simulink model "DWPUSH"  (R2026b)
settings: Solver=VariableStepAuto
undefined symbols (not defined in the file): Ac, Af, Ar, InitLinkage, Left, Linkage, Visual, X, Y, Z
libraries: sm_lib x57, Suspension_Utilities x43, nesl_utility x12, Linkage_Shock x1, fl_lib x1
(part 3 of 4)

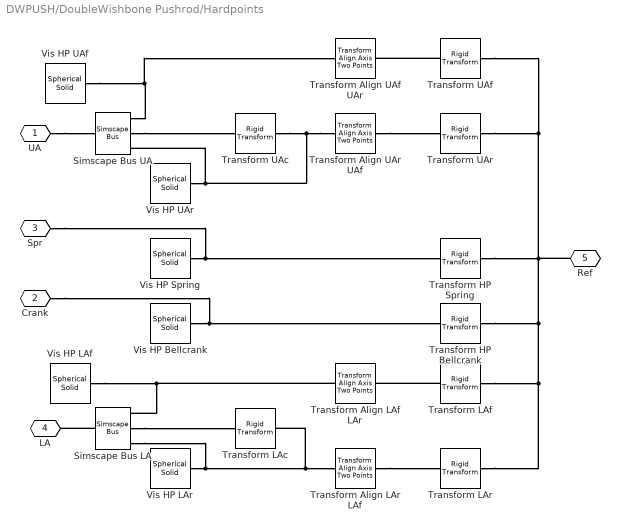
== system DWPUSH/DoubleWishbone Pushrod/Hardpoints ==
  Simscape Bus LA : SimscapeBus  HierarchyStrings=Af;Ac;Ar
  Simscape Bus UA : SimscapeBus  HierarchyStrings=Af;Ac;Ar
  Transform Align LAf LAr : Suspension_Utilities/Transform Align Axis Two Points  hp_b=hp_in_f_la.*rhs_hp  hp_t=hp_in_r_la.*rhs_hp  popup_f_axis=-Z
      settings: SourceProductName=SmCar - Suspension Utilites
  Transform Align LAr LAf : Suspension_Utilities/Transform Align Axis Two Points  hp_b=hp_in_r_la.*rhs_hp  hp_t=hp_in_f_la.*rhs_hp  popup_f_axis=+Z
      settings: SourceProductName=SmCar - Suspension Utilites
  Transform Align UAf UAr : Suspension_Utilities/Transform Align Axis Two Points  hp_b=hp_in_f_ua.*rhs_hp  hp_t=hp_in_r_ua.*rhs_hp  popup_f_axis=-Z
      settings: SourceProductName=SmCar - Suspension Utilites
  Transform Align UAr UAf : Suspension_Utilities/Transform Align Axis Two Points  hp_b=hp_in_r_ua.*rhs_hp  hp_t=hp_in_f_ua.*rhs_hp  popup_f_axis=+Z
      settings: SourceProductName=SmCar - Suspension Utilites
  Transform HP Bellcrank : sm_lib/Frames and Transforms/Rigid Transform  RotationMethod=None  FollAlignAxisA=+X  BaseAlignAxisA=+Y  FollAlignAxisB=+Y  BaseAlignAxisB=+Z  RotationStandardAxis=+Z  RotationAngle=0.0  RotationAngleUnits=deg  RotationArbitraryAxis=[0 0 1]  RotationSequenceAxes=FollowerAxes  RotationSequence=XYX  RotationSequenceAngles=[0 0 0]  RotationSequenceAnglesUnits=deg  RotationMatrix=[1 0 0; 0 1 0; 0 0 1]  Quaternion=[1 0 0 0]  TranslationMethod=Cartesian  TranslationCartesianOffset=hp_bellcrank.*rhs_hp  TranslationCartesianOffsetUnits=m  TranslationStandardAxis=+Z  TranslationStandardOffset=0  TranslationStandardOffsetUnits=m  TranslationROffset=0  TranslationROffsetUnits=m  TranslationThetaOffset=0  TranslationThetaOffsetUnits=deg  TranslationZOffset=0  TranslationZOffsetUnits=m
  Transform HP Spring : sm_lib/Frames and Transforms/Rigid Transform  RotationMethod=None  FollAlignAxisA=+X  BaseAlignAxisA=+Y  FollAlignAxisB=+Y  BaseAlignAxisB=+Z  RotationStandardAxis=+Z  RotationAngle=0.0  RotationAngleUnits=deg  RotationArbitraryAxis=[0 0 1]  RotationSequenceAxes=FollowerAxes  RotationSequence=XYX  RotationSequenceAngles=[0 0 0]  RotationSequenceAnglesUnits=deg  RotationMatrix=[1 0 0; 0 1 0; 0 0 1]  Quaternion=[1 0 0 0]  TranslationMethod=Cartesian  TranslationCartesianOffset=hp_spr_top.*rhs_hp  TranslationCartesianOffsetUnits=m  TranslationStandardAxis=+Z  TranslationStandardOffset=0  TranslationStandardOffsetUnits=m  TranslationROffset=0  TranslationROffsetUnits=m  TranslationThetaOffset=0  TranslationThetaOffsetUnits=deg  TranslationZOffset=0  TranslationZOffsetUnits=m
  Transform LAc : sm_lib/Frames and Transforms/Rigid Transform  RotationMethod=None  FollAlignAxisA=+X  BaseAlignAxisA=+Y  FollAlignAxisB=+Y  BaseAlignAxisB=+Z  RotationStandardAxis=+Z  RotationAngle=0  RotationAngleUnits=deg  RotationArbitraryAxis=[0 0 1]  RotationSequenceAxes=FollowerAxes  RotationSequence=XYX  RotationSequenceAngles=[0 0 0]  RotationSequenceAnglesUnits=deg  RotationMatrix=[0 0 -1;0 1 0;1 0 0]  Quaternion=[1 0 0 0]  TranslationMethod=StandardAxis  TranslationCartesianOffset=[0 0 0]  TranslationCartesianOffsetUnits=m  TranslationStandardAxis=+Z  TranslationStandardOffset=norm(hp_in_f_la-hp_in_r_la)/2  TranslationStandardOffsetUnits=m  TranslationROffset=0  TranslationROffsetUnits=m  TranslationThetaOffset=0  TranslationThetaOffsetUnits=deg  TranslationZOffset=0  TranslationZOffsetUnits=m
  Transform LAf : sm_lib/Frames and Transforms/Rigid Transform  RotationMethod=None  FollAlignAxisA=+X  BaseAlignAxisA=+Y  FollAlignAxisB=+Y  BaseAlignAxisB=+Z  RotationStandardAxis=+Z  RotationAngle=0.0  RotationAngleUnits=deg  RotationArbitraryAxis=[0 0 1]  RotationSequenceAxes=FollowerAxes  RotationSequence=XYX  RotationSequenceAngles=[0 0 0]  RotationSequenceAnglesUnits=deg  RotationMatrix=[1 0 0; 0 1 0; 0 0 1]  Quaternion=[1 0 0 0]  TranslationMethod=Cartesian  TranslationCartesianOffset=hp_in_f_la.*rhs_hp  TranslationCartesianOffsetUnits=m  TranslationStandardAxis=+Z  TranslationStandardOffset=0  TranslationStandardOffsetUnits=m  TranslationROffset=0  TranslationROffsetUnits=m  TranslationThetaOffset=0  TranslationThetaOffsetUnits=deg  TranslationZOffset=0  TranslationZOffsetUnits=m
  Transform LAr : sm_lib/Frames and Transforms/Rigid Transform  RotationMethod=None  FollAlignAxisA=+X  BaseAlignAxisA=+Y  FollAlignAxisB=+Y  BaseAlignAxisB=+Z  RotationStandardAxis=+Z  RotationAngle=0.0  RotationAngleUnits=deg  RotationArbitraryAxis=[0 0 1]  RotationSequenceAxes=FollowerAxes  RotationSequence=XYX  RotationSequenceAngles=[0 0 0]  RotationSequenceAnglesUnits=deg  RotationMatrix=[1 0 0; 0 1 0; 0 0 1]  Quaternion=[1 0 0 0]  TranslationMethod=Cartesian  TranslationCartesianOffset=hp_in_r_la.*rhs_hp  TranslationCartesianOffsetUnits=m  TranslationStandardAxis=+Z  TranslationStandardOffset=0  TranslationStandardOffsetUnits=m  TranslationROffset=0  TranslationROffsetUnits=m  TranslationThetaOffset=0  TranslationThetaOffsetUnits=deg  TranslationZOffset=0  TranslationZOffsetUnits=m
  Transform UAc : sm_lib/Frames and Transforms/Rigid Transform  RotationMethod=None  FollAlignAxisA=+X  BaseAlignAxisA=+Y  FollAlignAxisB=+Y  BaseAlignAxisB=+Z  RotationStandardAxis=+Z  RotationAngle=0  RotationAngleUnits=deg  RotationArbitraryAxis=[0 0 1]  RotationSequenceAxes=FollowerAxes  RotationSequence=XYX  RotationSequenceAngles=[0 0 0]  RotationSequenceAnglesUnits=deg  RotationMatrix=[0 0 -1;0 1 0;1 0 0]  Quaternion=[1 0 0 0]  TranslationMethod=StandardAxis  TranslationCartesianOffset=[0 0 0]  TranslationCartesianOffsetUnits=m  TranslationStandardAxis=+Z  TranslationStandardOffset=norm(hp_in_f_ua - hp_in_r_ua)/2  TranslationStandardOffsetUnits=m  TranslationROffset=0  TranslationROffsetUnits=m  TranslationThetaOffset=0  TranslationThetaOffsetUnits=deg  TranslationZOffset=0  TranslationZOffsetUnits=m
  Transform UAf : sm_lib/Frames and Transforms/Rigid Transform  RotationMethod=None  FollAlignAxisA=+X  BaseAlignAxisA=+Y  FollAlignAxisB=+Y  BaseAlignAxisB=+Z  RotationStandardAxis=+Z  RotationAngle=0.0  RotationAngleUnits=deg  RotationArbitraryAxis=[0 0 1]  RotationSequenceAxes=FollowerAxes  RotationSequence=XYX  RotationSequenceAngles=[0 0 0]  RotationSequenceAnglesUnits=deg  RotationMatrix=[1 0 0; 0 1 0; 0 0 1]  Quaternion=[1 0 0 0]  TranslationMethod=Cartesian  TranslationCartesianOffset=hp_in_f_ua.*rhs_hp  TranslationCartesianOffsetUnits=m  TranslationStandardAxis=+Z  TranslationStandardOffset=0  TranslationStandardOffsetUnits=m  TranslationROffset=0  TranslationROffsetUnits=m  TranslationThetaOffset=0  TranslationThetaOffsetUnits=deg  TranslationZOffset=0  TranslationZOffsetUnits=m
  Transform UAr : sm_lib/Frames and Transforms/Rigid Transform  RotationMethod=None  FollAlignAxisA=+X  BaseAlignAxisA=+Y  FollAlignAxisB=+Y  BaseAlignAxisB=+Z  RotationStandardAxis=+Z  RotationAngle=0.0  RotationAngleUnits=deg  RotationArbitraryAxis=[0 0 1]  RotationSequenceAxes=FollowerAxes  RotationSequence=XYX  RotationSequenceAngles=[0 0 0]  RotationSequenceAnglesUnits=deg  RotationMatrix=[1 0 0; 0 1 0; 0 0 1]  Quaternion=[1 0 0 0]  TranslationMethod=Cartesian  TranslationCartesianOffset=hp_in_r_ua.*rhs_hp  TranslationCartesianOffsetUnits=m  TranslationStandardAxis=+Z  TranslationStandardOffset=0  TranslationStandardOffsetUnits=m  TranslationROffset=0  TranslationROffsetUnits=m  TranslationThetaOffset=0  TranslationThetaOffsetUnits=deg  TranslationZOffset=0  TranslationZOffsetUnits=m
  Vis HP Bellcrank : sm_lib/Body Elements/Spherical Solid  SphereRadius=size_hp  SphereRadiusUnits=m  ExportEntireGeometry=off  InertiaType=CalculateFromGeometry  BasedOnType=Density  Density=0  DensityUnits=kg/m^3  Mass=1  MassUnits=kg  CenterOfMass=[0 0 0]  CenterOfMassUnits=m  MomentsOfInertia=[1 1 1]  MomentsOfInertiaUnits=kg*m^2  ProductsOfInertia=[0 0 0]  ProductsOfInertiaUnits=kg*m^2  GraphicType=FromGeometry  MarkerShape=Sphere  MarkerSize=10  GraphicVisPropType=SimpleVisualProperties  GraphicDiffuseColor=clr_hp  GraphicOpacity=opc_hp  GraphicSpecularColor=[0.5 0.5 0.5 1.0]  GraphicAmbientColor=[0.15 0.15 0.15 1.0]  GraphicEmissiveColor=[0.0 0.0 0.0 1.0]  GraphicShininess=75  DoExposeReferenceFrame=on  SerializedFrames=<Frames/>
  Vis HP LAf : sm_lib/Body Elements/Spherical Solid  SphereRadius=size_hp  SphereRadiusUnits=m  ExportEntireGeometry=off  InertiaType=CalculateFromGeometry  BasedOnType=Density  Density=0  DensityUnits=kg/m^3  Mass=1  MassUnits=kg  CenterOfMass=[0 0 0]  CenterOfMassUnits=m  MomentsOfInertia=[1 1 1]  MomentsOfInertiaUnits=kg*m^2  ProductsOfInertia=[0 0 0]  ProductsOfInertiaUnits=kg*m^2  GraphicType=FromGeometry  MarkerShape=Sphere  MarkerSize=10  GraphicVisPropType=SimpleVisualProperties  GraphicDiffuseColor=clr_hp  GraphicOpacity=opc_hp  GraphicSpecularColor=[0.5 0.5 0.5 1.0]  GraphicAmbientColor=[0.15 0.15 0.15 1.0]  GraphicEmissiveColor=[0.0 0.0 0.0 1.0]  GraphicShininess=75  DoExposeReferenceFrame=on  SerializedFrames=<Frames/>
  Vis HP LAr : sm_lib/Body Elements/Spherical Solid  SphereRadius=size_hp  SphereRadiusUnits=m  ExportEntireGeometry=off  InertiaType=CalculateFromGeometry  BasedOnType=Density  Density=0  DensityUnits=kg/m^3  Mass=1  MassUnits=kg  CenterOfMass=[0 0 0]  CenterOfMassUnits=m  MomentsOfInertia=[1 1 1]  MomentsOfInertiaUnits=kg*m^2  ProductsOfInertia=[0 0 0]  ProductsOfInertiaUnits=kg*m^2  GraphicType=FromGeometry  MarkerShape=Sphere  MarkerSize=10  GraphicVisPropType=SimpleVisualProperties  GraphicDiffuseColor=clr_hp  GraphicOpacity=opc_hp  GraphicSpecularColor=[0.5 0.5 0.5 1.0]  GraphicAmbientColor=[0.15 0.15 0.15 1.0]  GraphicEmissiveColor=[0.0 0.0 0.0 1.0]  GraphicShininess=75  DoExposeReferenceFrame=on  SerializedFrames=<Frames/>
  Vis HP Spring : sm_lib/Body Elements/Spherical Solid  SphereRadius=size_hp  SphereRadiusUnits=m  ExportEntireGeometry=off  InertiaType=CalculateFromGeometry  BasedOnType=Density  Density=0  DensityUnits=kg/m^3  Mass=1  MassUnits=kg  CenterOfMass=[0 0 0]  CenterOfMassUnits=m  MomentsOfInertia=[1 1 1]  MomentsOfInertiaUnits=kg*m^2  ProductsOfInertia=[0 0 0]  ProductsOfInertiaUnits=kg*m^2  GraphicType=FromGeometry  MarkerShape=Sphere  MarkerSize=10  GraphicVisPropType=SimpleVisualProperties  GraphicDiffuseColor=clr_hp  GraphicOpacity=opc_hp  GraphicSpecularColor=[0.5 0.5 0.5 1.0]  GraphicAmbientColor=[0.15 0.15 0.15 1.0]  GraphicEmissiveColor=[0.0 0.0 0.0 1.0]  GraphicShininess=75  DoExposeReferenceFrame=on  SerializedFrames=<Frames/>
  Vis HP UAf : sm_lib/Body Elements/Spherical Solid  SphereRadius=size_hp  SphereRadiusUnits=m  ExportEntireGeometry=off  InertiaType=CalculateFromGeometry  BasedOnType=Density  Density=0  DensityUnits=kg/m^3  Mass=1  MassUnits=kg  CenterOfMass=[0 0 0]  CenterOfMassUnits=m  MomentsOfInertia=[1 1 1]  MomentsOfInertiaUnits=kg*m^2  ProductsOfInertia=[0 0 0]  ProductsOfInertiaUnits=kg*m^2  GraphicType=FromGeometry  MarkerShape=Sphere  MarkerSize=10  GraphicVisPropType=SimpleVisualProperties  GraphicDiffuseColor=clr_hp  GraphicOpacity=opc_hp  GraphicSpecularColor=[0.5 0.5 0.5 1.0]  GraphicAmbientColor=[0.15 0.15 0.15 1.0]  GraphicEmissiveColor=[0.0 0.0 0.0 1.0]  GraphicShininess=75  DoExposeReferenceFrame=on  SerializedFrames=<Frames/>
  Vis HP UAr : sm_lib/Body Elements/Spherical Solid  SphereRadius=size_hp  SphereRadiusUnits=m  ExportEntireGeometry=off  InertiaType=CalculateFromGeometry  BasedOnType=Density  Density=0  DensityUnits=kg/m^3  Mass=1  MassUnits=kg  CenterOfMass=[0 0 0]  CenterOfMassUnits=m  MomentsOfInertia=[1 1 1]  MomentsOfInertiaUnits=kg*m^2  ProductsOfInertia=[0 0 0]  ProductsOfInertiaUnits=kg*m^2  GraphicType=FromGeometry  MarkerShape=Sphere  MarkerSize=10  GraphicVisPropType=SimpleVisualProperties  GraphicDiffuseColor=clr_hp  GraphicOpacity=opc_hp  GraphicSpecularColor=[0.5 0.5 0.5 1.0]  GraphicAmbientColor=[0.15 0.15 0.15 1.0]  GraphicEmissiveColor=[0.0 0.0 0.0 1.0]  GraphicShininess=75  DoExposeReferenceFrame=on  SerializedFrames=<Frames/>
  UA : PMIOPort  Side=Left
  Crank : PMIOPort  Port=2  Side=Left
  Spr : PMIOPort  Port=3  Side=Left
  LA : PMIOPort  Port=4  Side=Left
  Ref : PMIOPort  Port=5  Side=Right
  connections:
  Transform LAf/RConn1 -- Transform Align LAf LAr/LConn1
  Transform Align LAr LAf/LConn1 -- Transform LAr/RConn1
  Transform Align UAr UAf/RConn1 -- Vis HP UAr/RConn1 -- Simscape Bus UA/LConn3 -- Transform UAc/LConn1
  Transform Align UAr UAf/LConn1 -- Transform UAr/RConn1
  Transform UAf/RConn1 -- Transform Align UAf UAr/LConn1
  Vis HP Spring/RConn1 -- Spr/RConn1 -- Transform HP Spring/RConn1
  Simscape Bus UA/LConn1 -- Vis HP UAf/RConn1 -- Transform Align UAf UAr/RConn1
  Vis HP LAr/RConn1 -- Transform Align LAr LAf/RConn1 -- Transform LAc/LConn1 -- Simscape Bus LA/LConn3
  Vis HP LAf/RConn1 -- Transform Align LAf LAr/RConn1 -- Simscape Bus LA/LConn1
  Ref/RConn1 -- Transform HP Spring/LConn1 -- Transform UAr/LConn1 -- Transform UAf/LConn1 -- Transform HP Bellcrank/LConn1 -- Transform LAf/LConn1 -- Transform LAr/LConn1
  Simscape Bus UA/LConn2 -- Transform UAc/RConn1
  UA/RConn1 -- Simscape Bus UA/RConn1
  Simscape Bus LA/LConn2 -- Transform LAc/RConn1
  Simscape Bus LA/RConn1 -- LA/RConn1
  Vis HP Bellcrank/RConn1 -- Crank/RConn1 -- Transform HP Bellcrank/RConn1

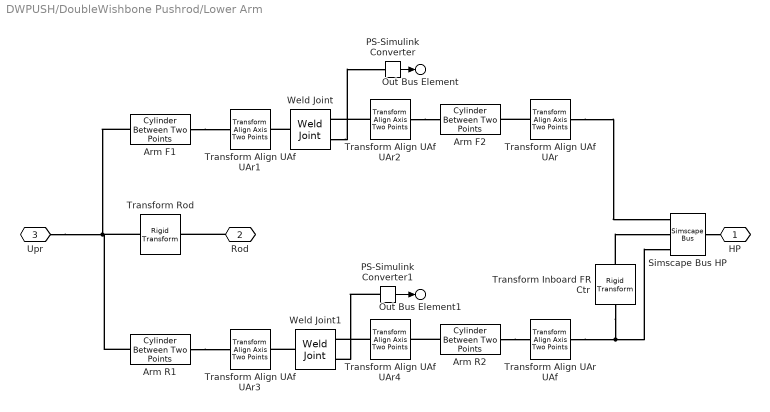
== system DWPUSH/DoubleWishbone Pushrod/Lower Arm ==
  Arm F1 : Suspension_Utilities/Cylinder Between Two Points  hp_b=hp_rod_f.*rhs_hp  hp_f=hp_out.*rhs_hp  Mass=la_mass/2  clr_solid=clr_solid  opc_solid=opc_solid  rad_solid=rad_solid
      settings: SourceProductName=SmCar - Suspension Utilites
  Arm F2 : Suspension_Utilities/Cylinder Between Two Points  hp_b=hp_rod_f.*rhs_hp  hp_f=hp_out.*rhs_hp  Mass=la_mass/2  clr_solid=clr_solid  opc_solid=opc_solid  rad_solid=rad_solid
      settings: SourceProductName=SmCar - Suspension Utilites
  Arm R1 : Suspension_Utilities/Cylinder Between Two Points  hp_b=hp_rod_r.*rhs_hp  hp_f=hp_out.*rhs_hp  Mass=ua_mass/4  clr_solid=clr_solid  opc_solid=opc_solid  rad_solid=rad_solid
      settings: SourceProductName=SmCar - Suspension Utilites
  Arm R2 : Suspension_Utilities/Cylinder Between Two Points  hp_b=hp_in_r.*rhs_hp  hp_f=hp_rod_r.*rhs_hp  Mass=ua_mass/4  clr_solid=clr_solid  opc_solid=opc_solid  rad_solid=rad_solid
      settings: SourceProductName=SmCar - Suspension Utilites
  PS-Simulink Converter : nesl_utility/PS-Simulink Converter  PhysicalDomain=network_engine_domain  SubClassName=ps_output  LeftPortType=input  RightPortType=output  PseudoPeriodic=off  Frequencies=[]  VectorFormat=inherit  Unit=inherit  AffineConversion=off
  PS-Simulink Converter1 : nesl_utility/PS-Simulink Converter  PhysicalDomain=network_engine_domain  SubClassName=ps_output  LeftPortType=input  RightPortType=output  PseudoPeriodic=off  Frequencies=[]  VectorFormat=inherit  Unit=inherit  AffineConversion=off
  Simscape Bus HP : SimscapeBus  HierarchyStrings=Af;Ac;Ar
  Transform Align UAf UAr : Suspension_Utilities/Transform Align Axis Two Points  hp_b=hp_in_r.*rhs_hp  hp_t=hp_in_f.*rhs_hp  popup_f_axis=+Z
      settings: SourceProductName=SmCar - Suspension Utilites
  Transform Align UAf UAr1 : Suspension_Utilities/Transform Align Axis Two Points  hp_b=hp_rod_f.*rhs_hp  hp_t=hp_in_f.*rhs_hp  popup_f_axis=+Y
      settings: SourceProductName=SmCar - Suspension Utilites
  Transform Align UAf UAr2 : Suspension_Utilities/Transform Align Axis Two Points  hp_b=hp_rod_f.*rhs_hp  hp_t=hp_in_f.*rhs_hp  popup_f_axis=+Y
      settings: SourceProductName=SmCar - Suspension Utilites
  Transform Align UAf UAr3 : Suspension_Utilities/Transform Align Axis Two Points  hp_b=hp_rod_r.*rhs_hp  hp_t=hp_in_r.*rhs_hp  popup_f_axis=+Y
      settings: SourceProductName=SmCar - Suspension Utilites
  Transform Align UAf UAr4 : Suspension_Utilities/Transform Align Axis Two Points  hp_b=hp_rod_r.*rhs_hp  hp_t=hp_in_r.*rhs_hp  popup_f_axis=+Y
      settings: SourceProductName=SmCar - Suspension Utilites
  Transform Align UAr UAf : Suspension_Utilities/Transform Align Axis Two Points  hp_b=hp_in_r.*rhs_hp  hp_t=hp_in_f.*rhs_hp  popup_f_axis=+Z
      settings: SourceProductName=SmCar - Suspension Utilites
  Transform Inboard FR Ctr : sm_lib/Frames and Transforms/Rigid Transform  RotationMethod=None  FollAlignAxisA=+X  BaseAlignAxisA=+Y  FollAlignAxisB=+Y  BaseAlignAxisB=+Z  RotationStandardAxis=+Z  RotationAngle=0.0  RotationAngleUnits=deg  RotationArbitraryAxis=[0 0 1]  RotationSequenceAxes=FollowerAxes  RotationSequence=XYX  RotationSequenceAngles=[0 0 0]  RotationSequenceAnglesUnits=deg  RotationMatrix=[1 0 0; 0 1 0; 0 0 1]  Quaternion=[1 0 0 0]  TranslationMethod=StandardAxis  TranslationCartesianOffset=[0 0 0]  TranslationCartesianOffsetUnits=m  TranslationStandardAxis=+Z  TranslationStandardOffset=norm(hp_in_f-hp_in_r)/2  TranslationStandardOffsetUnits=m  TranslationROffset=0  TranslationROffsetUnits=m  TranslationThetaOffset=0  TranslationThetaOffsetUnits=deg  TranslationZOffset=0  TranslationZOffsetUnits=m
  Transform Rod : sm_lib/Frames and Transforms/Rigid Transform  RotationMethod=None  FollAlignAxisA=+X  BaseAlignAxisA=+Y  FollAlignAxisB=+Y  BaseAlignAxisB=+Z  RotationStandardAxis=+Z  RotationAngle=0.0  RotationAngleUnits=deg  RotationArbitraryAxis=[0 0 1]  RotationSequenceAxes=FollowerAxes  RotationSequence=XYX  RotationSequenceAngles=[0 0 0]  RotationSequenceAnglesUnits=deg  RotationMatrix=[1 0 0; 0 1 0; 0 0 1]  Quaternion=[1 0 0 0]  TranslationMethod=Cartesian  TranslationCartesianOffset=(hp_rod-hp_out).*rhs_hp  TranslationCartesianOffsetUnits=m  TranslationStandardAxis=+Z  TranslationStandardOffset=0  TranslationStandardOffsetUnits=m  TranslationROffset=0  TranslationROffsetUnits=m  TranslationThetaOffset=0  TranslationThetaOffsetUnits=deg  TranslationZOffset=0  TranslationZOffsetUnits=m
  Weld Joint : sm_lib/Joints/Weld Joint  JointMode=Normal  CompositeWrenchDir=FollowerOnBase  CompositeWrenchFrame=BaseFrame  SenseConstraintForce=off  SenseConstraintTorque=off  SenseTotalForce=on  SenseTotalTorque=off
  Weld Joint1 : sm_lib/Joints/Weld Joint  JointMode=Normal  CompositeWrenchDir=FollowerOnBase  CompositeWrenchFrame=BaseFrame  SenseConstraintForce=off  SenseConstraintTorque=off  SenseTotalForce=on  SenseTotalTorque=off
  HP : PMIOPort  Side=Right
  Rod : PMIOPort  Port=2  Side=Left
  Upr : PMIOPort  Port=3  Side=Left
  Out Bus Element : Outport  PortName=m  Element=Front
  Out Bus Element1 : Outport  PortName=m  Element=Rear
  wires:
  PS-Simulink Converter/1 -> Out Bus Element/1
  PS-Simulink Converter1/1 -> Out Bus Element1/1
  connections:
  Rod/RConn1 -- Transform Rod/RConn1
  Transform Align UAf UAr/RConn1 -- Simscape Bus HP/LConn1
  Transform Align UAf UAr/LConn1 -- Arm F2/LConn1
  Arm R2/LConn1 -- Transform Align UAr UAf/LConn1
  Simscape Bus HP/RConn1 -- HP/RConn1
  Transform Inboard FR Ctr/RConn1 -- Simscape Bus HP/LConn2
  Transform Inboard FR Ctr/LConn1 -- Simscape Bus HP/LConn3 -- Transform Align UAr UAf/RConn1
  Arm F1/RConn1 -- Arm R1/RConn1 -- Transform Rod/LConn1 -- Upr/RConn1
  Arm F1/LConn1 -- Transform Align UAf UAr1/LConn1
  Transform Align UAf UAr2/RConn1 -- Weld Joint/RConn1
  Weld Joint/LConn1 -- Transform Align UAf UAr1/RConn1
  Weld Joint/RConn2 -- PS-Simulink Converter/LConn1
  Transform Align UAf UAr2/LConn1 -- Arm F2/RConn1
  Arm R1/LConn1 -- Transform Align UAf UAr3/LConn1
  Transform Align UAf UAr4/RConn1 -- Weld Joint1/RConn1
  Weld Joint1/LConn1 -- Transform Align UAf UAr3/RConn1
  Arm R2/RConn1 -- Transform Align UAf UAr4/LConn1
  PS-Simulink Converter1/LConn1 -- Weld Joint1/RConn2

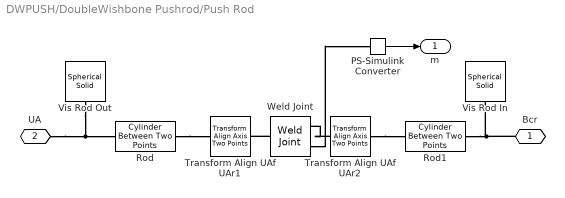
== system DWPUSH/DoubleWishbone Pushrod/Push Rod ==
  PS-Simulink Converter : nesl_utility/PS-Simulink Converter  PhysicalDomain=network_engine_domain  SubClassName=ps_output  LeftPortType=input  RightPortType=output  PseudoPeriodic=off  Frequencies=[]  VectorFormat=inherit  Unit=inherit  AffineConversion=off
  Rod : Suspension_Utilities/Cylinder Between Two Points  hp_b=hp_rod_c.*rhs_hp  hp_f=hp_out.*rhs_hp  Mass=rod_mass/2  clr_solid=clr_rod  opc_solid=opc_rod  rad_solid=radius_rod
      settings: SourceProductName=SmCar - Suspension Utilites
  Rod1 : Suspension_Utilities/Cylinder Between Two Points  hp_b=hp_rod_c.*rhs_hp  hp_f=hp_out.*rhs_hp  Mass=rod_mass/2  clr_solid=clr_rod  opc_solid=opc_rod  rad_solid=radius_rod
      settings: SourceProductName=SmCar - Suspension Utilites
  Transform Align UAf UAr1 : Suspension_Utilities/Transform Align Axis Two Points  hp_b=hp_rod_c.*rhs_hp  hp_t=hp_in.*rhs_hp  popup_f_axis=-Z
      settings: SourceProductName=SmCar - Suspension Utilites
  Transform Align UAf UAr2 : Suspension_Utilities/Transform Align Axis Two Points  hp_b=hp_rod_c.*rhs_hp  hp_t=hp_in.*rhs_hp  popup_f_axis=-Z
      settings: SourceProductName=SmCar - Suspension Utilites
  Vis Rod In : sm_lib/Body Elements/Spherical Solid  SphereRadius=size_conn_rod  SphereRadiusUnits=m  ExportEntireGeometry=off  InertiaType=CalculateFromGeometry  BasedOnType=Density  Density=0  DensityUnits=kg/m^3  Mass=1  MassUnits=kg  CenterOfMass=[0 0 0]  CenterOfMassUnits=m  MomentsOfInertia=[1 1 1]  MomentsOfInertiaUnits=kg*m^2  ProductsOfInertia=[0 0 0]  ProductsOfInertiaUnits=kg*m^2  GraphicType=FromGeometry  MarkerShape=Sphere  MarkerSize=10  GraphicVisPropType=SimpleVisualProperties  GraphicDiffuseColor=clr_conn_rod  GraphicOpacity=opc_conn_rod  GraphicSpecularColor=[0.5 0.5 0.5 1.0]  GraphicAmbientColor=[0.15 0.15 0.15 1.0]  GraphicEmissiveColor=[0.0 0.0 0.0 1.0]  GraphicShininess=75  DoExposeReferenceFrame=on  SerializedFrames=<Frames/>
  Vis Rod Out : sm_lib/Body Elements/Spherical Solid  SphereRadius=size_conn_rod  SphereRadiusUnits=m  ExportEntireGeometry=off  InertiaType=CalculateFromGeometry  BasedOnType=Density  Density=0  DensityUnits=kg/m^3  Mass=1  MassUnits=kg  CenterOfMass=[0 0 0]  CenterOfMassUnits=m  MomentsOfInertia=[1 1 1]  MomentsOfInertiaUnits=kg*m^2  ProductsOfInertia=[0 0 0]  ProductsOfInertiaUnits=kg*m^2  GraphicType=FromGeometry  MarkerShape=Sphere  MarkerSize=10  GraphicVisPropType=SimpleVisualProperties  GraphicDiffuseColor=clr_conn_rod  GraphicOpacity=opc_conn_rod  GraphicSpecularColor=[0.5 0.5 0.5 1.0]  GraphicAmbientColor=[0.15 0.15 0.15 1.0]  GraphicEmissiveColor=[0.0 0.0 0.0 1.0]  GraphicShininess=75  DoExposeReferenceFrame=on  SerializedFrames=<Frames/>
  Weld Joint : sm_lib/Joints/Weld Joint  JointMode=Normal  CompositeWrenchDir=FollowerOnBase  CompositeWrenchFrame=BaseFrame  SenseConstraintForce=off  SenseConstraintTorque=off  SenseTotalForce=on  SenseTotalTorque=off
  Bcr : PMIOPort  Side=Right
  UA : PMIOPort  Port=2  Side=Left
  m : Outport
  wires:
  PS-Simulink Converter/1 -> m/1
  connections:
  UA/RConn1 -- Rod/RConn1 -- Vis Rod Out/RConn1
  Rod1/LConn1 -- Vis Rod In/RConn1 -- Bcr/RConn1
  Transform Align UAf UAr2/RConn1 -- Weld Joint/RConn1
  Weld Joint/LConn1 -- Transform Align UAf UAr1/RConn1
  Rod/LConn1 -- Transform Align UAf UAr1/LConn1
  Transform Align UAf UAr2/LConn1 -- Rod1/RConn1
  Weld Joint/RConn2 -- PS-Simulink Converter/LConn1

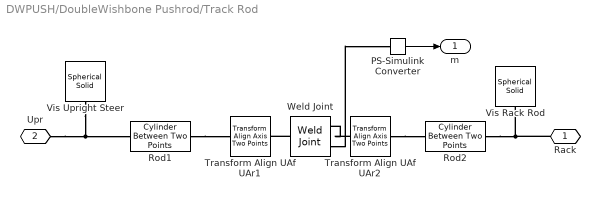
== system DWPUSH/DoubleWishbone Pushrod/Track Rod ==
  PS-Simulink Converter : nesl_utility/PS-Simulink Converter  PhysicalDomain=network_engine_domain  SubClassName=ps_output  LeftPortType=input  RightPortType=output  PseudoPeriodic=off  Frequencies=[]  VectorFormat=inherit  Unit=inherit  AffineConversion=off
  Rod1 : Suspension_Utilities/Cylinder Between Two Points  hp_b=hp_rod_c.*rhs_hp  hp_f=hp_out.*rhs_hp  Mass=rod_mass/2  clr_solid=clr_rod  opc_solid=opc_rod  rad_solid=radius_rod
      settings: SourceProductName=SmCar - Suspension Utilites
  Rod2 : Suspension_Utilities/Cylinder Between Two Points  hp_b=hp_rod_c.*rhs_hp  hp_f=hp_out.*rhs_hp  Mass=rod_mass/2  clr_solid=clr_rod  opc_solid=opc_rod  rad_solid=radius_rod
      settings: SourceProductName=SmCar - Suspension Utilites
  Transform Align UAf UAr1 : Suspension_Utilities/Transform Align Axis Two Points  hp_b=hp_rod_c.*rhs_hp  hp_t=hp_in.*rhs_hp  popup_f_axis=-Z
      settings: SourceProductName=SmCar - Suspension Utilites
  Transform Align UAf UAr2 : Suspension_Utilities/Transform Align Axis Two Points  hp_b=hp_rod_c.*rhs_hp  hp_t=hp_in.*rhs_hp  popup_f_axis=-Z
      settings: SourceProductName=SmCar - Suspension Utilites
  Vis Rack Rod : sm_lib/Body Elements/Spherical Solid  SphereRadius=size_conn_rod  SphereRadiusUnits=m  ExportEntireGeometry=off  InertiaType=CalculateFromGeometry  BasedOnType=Density  Density=0  DensityUnits=kg/m^3  Mass=1  MassUnits=kg  CenterOfMass=[0 0 0]  CenterOfMassUnits=m  MomentsOfInertia=[1 1 1]  MomentsOfInertiaUnits=kg*m^2  ProductsOfInertia=[0 0 0]  ProductsOfInertiaUnits=kg*m^2  GraphicType=FromGeometry  MarkerShape=Sphere  MarkerSize=10  GraphicVisPropType=SimpleVisualProperties  GraphicDiffuseColor=clr_conn_rod  GraphicOpacity=opc_conn_rod  GraphicSpecularColor=[0.5 0.5 0.5 1.0]  GraphicAmbientColor=[0.15 0.15 0.15 1.0]  GraphicEmissiveColor=[0.0 0.0 0.0 1.0]  GraphicShininess=75  DoExposeReferenceFrame=on  SerializedFrames=<Frames/>
  Vis Upright Steer : sm_lib/Body Elements/Spherical Solid  SphereRadius=size_conn_rod  SphereRadiusUnits=m  ExportEntireGeometry=off  InertiaType=CalculateFromGeometry  BasedOnType=Density  Density=0  DensityUnits=kg/m^3  Mass=1  MassUnits=kg  CenterOfMass=[0 0 0]  CenterOfMassUnits=m  MomentsOfInertia=[1 1 1]  MomentsOfInertiaUnits=kg*m^2  ProductsOfInertia=[0 0 0]  ProductsOfInertiaUnits=kg*m^2  GraphicType=FromGeometry  MarkerShape=Sphere  MarkerSize=10  GraphicVisPropType=SimpleVisualProperties  GraphicDiffuseColor=clr_conn_rod  GraphicOpacity=opc_conn_rod  GraphicSpecularColor=[0.5 0.5 0.5 1.0]  GraphicAmbientColor=[0.15 0.15 0.15 1.0]  GraphicEmissiveColor=[0.0 0.0 0.0 1.0]  GraphicShininess=75  DoExposeReferenceFrame=on  SerializedFrames=<Frames/>
  Weld Joint : sm_lib/Joints/Weld Joint  JointMode=Normal  CompositeWrenchDir=FollowerOnBase  CompositeWrenchFrame=BaseFrame  SenseConstraintForce=off  SenseConstraintTorque=off  SenseTotalForce=on  SenseTotalTorque=off
  Rack : PMIOPort  Side=Right
  Upr : PMIOPort  Port=2  Side=Left
  m : Outport
  wires:
  PS-Simulink Converter/1 -> m/1
  connections:
  Vis Upright Steer/RConn1 -- Rod1/RConn1 -- Upr/RConn1
  Rack/RConn1 -- Rod2/LConn1 -- Vis Rack Rod/RConn1
  Weld Joint/RConn2 -- PS-Simulink Converter/LConn1
  Weld Joint/LConn1 -- Transform Align UAf UAr1/RConn1
  Rod1/LConn1 -- Transform Align UAf UAr1/LConn1
  Transform Align UAf UAr2/RConn1 -- Weld Joint/RConn1
  Transform Align UAf UAr2/LConn1 -- Rod2/RConn1

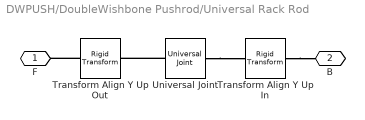
== system DWPUSH/DoubleWishbone Pushrod/Universal Rack Rod ==
  Transform Align Y Up In : sm_lib/Frames and Transforms/Rigid Transform  RotationMethod=StandardAxis  FollAlignAxisA=+X  BaseAlignAxisA=+Y  FollAlignAxisB=+Y  BaseAlignAxisB=+Z  RotationStandardAxis=+X  RotationAngle=90  RotationAngleUnits=deg  RotationArbitraryAxis=[0 0 1]  RotationSequenceAxes=FollowerAxes  RotationSequence=XYX  RotationSequenceAngles=[0 0 0]  RotationSequenceAnglesUnits=deg  RotationMatrix=[1 0 0; 0 1 0; 0 0 1]  Quaternion=[1 0 0 0]  TranslationMethod=None  TranslationCartesianOffset=[0 0 0]  TranslationCartesianOffsetUnits=m  TranslationStandardAxis=+Z  TranslationStandardOffset=0  TranslationStandardOffsetUnits=m  TranslationROffset=0  TranslationROffsetUnits=m  TranslationThetaOffset=0  TranslationThetaOffsetUnits=deg  TranslationZOffset=0  TranslationZOffsetUnits=m
  Transform Align Y Up Out : sm_lib/Frames and Transforms/Rigid Transform  RotationMethod=StandardAxis  FollAlignAxisA=+X  BaseAlignAxisA=+Y  FollAlignAxisB=+Y  BaseAlignAxisB=+Z  RotationStandardAxis=+X  RotationAngle=90  RotationAngleUnits=deg  RotationArbitraryAxis=[0 0 1]  RotationSequenceAxes=FollowerAxes  RotationSequence=XYX  RotationSequenceAngles=[0 0 0]  RotationSequenceAnglesUnits=deg  RotationMatrix=[1 0 0; 0 1 0; 0 0 1]  Quaternion=[1 0 0 0]  TranslationMethod=None  TranslationCartesianOffset=[0 0 0]  TranslationCartesianOffsetUnits=m  TranslationStandardAxis=+Z  TranslationStandardOffset=0  TranslationStandardOffsetUnits=m  TranslationROffset=0  TranslationROffsetUnits=m  TranslationThetaOffset=0  TranslationThetaOffsetUnits=deg  TranslationZOffset=0  TranslationZOffsetUnits=m
  Universal Joint : sm_lib/Joints/Universal Joint  JointMode=Normal  CompositeWrenchDir=FollowerOnBase  CompositeWrenchFrame=BaseFrame  SenseConstraintForce=off  SenseConstraintTorque=off  SenseTotalForce=off  SenseTotalTorque=off  RxPositionTargetSpecify=off  RxPositionTargetPriority=Low  RxPositionTargetValue=0  RxPositionTargetValueUnits=deg  RxVelocityTargetSpecify=off  RxVelocityTargetPriority=High  RxVelocityTargetValue=0  RxVelocityTargetValueUnits=deg/s  RxEquilibriumPosition=0  RxEquilibriumPositionUnits=deg  RxSpringStiffness=0  RxSpringStiffnessUnits=N*m/deg  RxDampingCoefficient=0  RxDampingCoefficientUnits=N*m/(deg/s)  RxLowerLimitSpecify=off  RxLowerLimitBound=-90  RxLowerLimitBoundUnits=deg  RxLowerLimitStiffness=1e4  RxLowerLimitStiffnessUnits=N*m/deg  RxLowerLimitDamping=10  RxLowerLimitDampingUnits=N*m/(deg/s)  RxLowerLimitTransitionRegionWidth=0.1  RxLowerLimitTransitionRegionWidthUnits=deg  RxUpperLimitSpecify=off  RxUpperLimitBound=90  RxUpperLimitBoundUnits=deg  RxUpperLimitStiffness=1e4  RxUpperLimitStiffnessUnits=N*m/deg  RxUpperLimitDamping=10  RxUpperLimitDampingUnits=N*m/(deg/s)  RxUpperLimitTransitionRegionWidth=0.1  RxUpperLimitTransitionRegionWidthUnits=deg  RxTorqueActuationMode=NoTorque  RxMotionActuationMode=ComputedMotion  RxSensePosition=off  RxSenseVelocity=off  RxSenseAcceleration=off  RxSenseTorqueForce=off  RxSenseLowerLimitTorqueForce=off  RxSenseUpperLimitTorqueForce=off  RyPositionTargetSpecify=off  RyPositionTargetPriority=High  RyPositionTargetValue=0  RyPositionTargetValueUnits=deg  RyVelocityTargetSpecify=off  RyVelocityTargetPriority=High  RyVelocityTargetValue=0  RyVelocityTargetValueUnits=deg/s  RyEquilibriumPosition=0  RyEquilibriumPositionUnits=deg  RySpringStiffness=0  RySpringStiffnessUnits=N*m/deg  RyDampingCoefficient=0  RyDampingCoefficientUnits=N*m/(deg/s)  RyLowerLimitSpecify=off  RyLowerLimitBound=-90  RyLowerLimitBoundUnits=deg  RyLowerLimitStiffness=1e4  RyLowerLimitStiffnessUnits=N*m/deg  RyLowerLimitDamping=10  RyLowerLimitDampingUnits=N*m/(deg/s)  RyLowerLimitTransitionRegionWidth=0.1  RyLowerLimitTransitionRegionWidthUnits=deg  RyUpperLimitSpecify=off  RyUpperLimitBound=90  RyUpperLimitBoundUnits=deg  RyUpperLimitStiffness=1e4  RyUpperLimitStiffnessUnits=N*m/deg  RyUpperLimitDamping=10  RyUpperLimitDampingUnits=N*m/(deg/s)  RyUpperLimitTransitionRegionWidth=0.1  RyUpperLimitTransitionRegionWidthUnits=deg  RyTorqueActuationMode=NoTorque  RyMotionActuationMode=ComputedMotion  RySensePosition=off  RySenseVelocity=off  RySenseAcceleration=off  RySenseTorqueForce=off  RySenseLowerLimitTorqueForce=off  RySenseUpperLimitTorqueForce=off
  F : PMIOPort  Side=Left
  B : PMIOPort  Port=2  Side=Right
  connections:
  Universal Joint/RConn1 -- Transform Align Y Up Out/RConn1
  Transform Align Y Up In/LConn1 -- B/RConn1
  Universal Joint/LConn1 -- Transform Align Y Up In/RConn1
  Transform Align Y Up Out/LConn1 -- F/RConn1

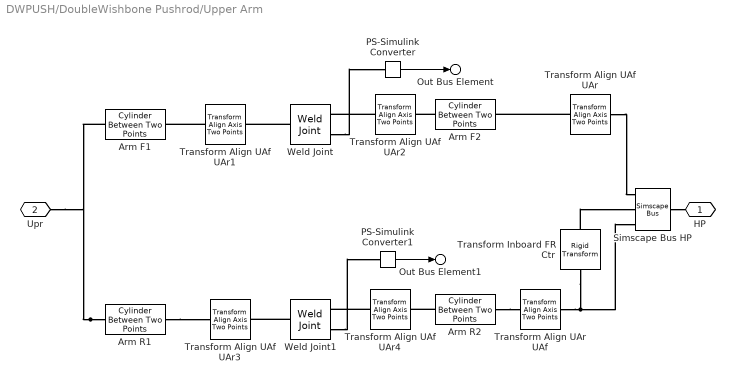
== system DWPUSH/DoubleWishbone Pushrod/Upper Arm ==
  Arm F1 : Suspension_Utilities/Cylinder Between Two Points  hp_b=hp_rod_f.*rhs_hp  hp_f=hp_out.*rhs_hp  Mass=ua_mass/4  clr_solid=clr_solid  opc_solid=opc_solid  rad_solid=rad_solid
      settings: SourceProductName=SmCar - Suspension Utilites
  Arm F2 : Suspension_Utilities/Cylinder Between Two Points  hp_b=hp_in_f.*rhs_hp  hp_f=hp_rod_f.*rhs_hp  Mass=ua_mass/4  clr_solid=clr_solid  opc_solid=opc_solid  rad_solid=rad_solid
      settings: SourceProductName=SmCar - Suspension Utilites
  Arm R1 : Suspension_Utilities/Cylinder Between Two Points  hp_b=hp_rod_r.*rhs_hp  hp_f=hp_out.*rhs_hp  Mass=ua_mass/4  clr_solid=clr_solid  opc_solid=opc_solid  rad_solid=rad_solid
      settings: SourceProductName=SmCar - Suspension Utilites
  Arm R2 : Suspension_Utilities/Cylinder Between Two Points  hp_b=hp_in_r.*rhs_hp  hp_f=hp_rod_r.*rhs_hp  Mass=ua_mass/4  clr_solid=clr_solid  opc_solid=opc_solid  rad_solid=rad_solid
      settings: SourceProductName=SmCar - Suspension Utilites
  PS-Simulink Converter : nesl_utility/PS-Simulink Converter  PhysicalDomain=network_engine_domain  SubClassName=ps_output  LeftPortType=input  RightPortType=output  PseudoPeriodic=off  Frequencies=[]  VectorFormat=inherit  Unit=inherit  AffineConversion=off
  PS-Simulink Converter1 : nesl_utility/PS-Simulink Converter  PhysicalDomain=network_engine_domain  SubClassName=ps_output  LeftPortType=input  RightPortType=output  PseudoPeriodic=off  Frequencies=[]  VectorFormat=inherit  Unit=inherit  AffineConversion=off
  Simscape Bus HP : SimscapeBus  HierarchyStrings=Af;Ac;Ar
  Transform Align UAf UAr : Suspension_Utilities/Transform Align Axis Two Points  hp_b=hp_in_r.*rhs_hp  hp_t=hp_in_f.*rhs_hp  popup_f_axis=+Z
      settings: SourceProductName=SmCar - Suspension Utilites
  Transform Align UAf UAr1 : Suspension_Utilities/Transform Align Axis Two Points  hp_b=hp_rod_f.*rhs_hp  hp_t=hp_in_f.*rhs_hp  popup_f_axis=+Y
      settings: SourceProductName=SmCar - Suspension Utilites
  Transform Align UAf UAr2 : Suspension_Utilities/Transform Align Axis Two Points  hp_b=hp_rod_f.*rhs_hp  hp_t=hp_in_f.*rhs_hp  popup_f_axis=+Y
      settings: SourceProductName=SmCar - Suspension Utilites
  Transform Align UAf UAr3 : Suspension_Utilities/Transform Align Axis Two Points  hp_b=hp_rod_r.*rhs_hp  hp_t=hp_in_r.*rhs_hp  popup_f_axis=+Y
      settings: SourceProductName=SmCar - Suspension Utilites
  Transform Align UAf UAr4 : Suspension_Utilities/Transform Align Axis Two Points  hp_b=hp_rod_r.*rhs_hp  hp_t=hp_in_r.*rhs_hp  popup_f_axis=+Y
      settings: SourceProductName=SmCar - Suspension Utilites
  Transform Align UAr UAf : Suspension_Utilities/Transform Align Axis Two Points  hp_b=hp_in_r.*rhs_hp  hp_t=hp_in_f.*rhs_hp  popup_f_axis=+Z
      settings: SourceProductName=SmCar - Suspension Utilites
  Transform Inboard FR Ctr : sm_lib/Frames and Transforms/Rigid Transform  RotationMethod=None  FollAlignAxisA=+X  BaseAlignAxisA=+Y  FollAlignAxisB=+Y  BaseAlignAxisB=+Z  RotationStandardAxis=+Z  RotationAngle=0.0  RotationAngleUnits=deg  RotationArbitraryAxis=[0 0 1]  RotationSequenceAxes=FollowerAxes  RotationSequence=XYX  RotationSequenceAngles=[0 0 0]  RotationSequenceAnglesUnits=deg  RotationMatrix=[1 0 0; 0 1 0; 0 0 1]  Quaternion=[1 0 0 0]  TranslationMethod=StandardAxis  TranslationCartesianOffset=[0 0 0]  TranslationCartesianOffsetUnits=m  TranslationStandardAxis=+Z  TranslationStandardOffset=norm(hp_in_f-hp_in_r)/2  TranslationStandardOffsetUnits=m  TranslationROffset=0  TranslationROffsetUnits=m  TranslationThetaOffset=0  TranslationThetaOffsetUnits=deg  TranslationZOffset=0  TranslationZOffsetUnits=m
  Weld Joint : sm_lib/Joints/Weld Joint  JointMode=Normal  CompositeWrenchDir=FollowerOnBase  CompositeWrenchFrame=BaseFrame  SenseConstraintForce=off  SenseConstraintTorque=off  SenseTotalForce=on  SenseTotalTorque=off
  Weld Joint1 : sm_lib/Joints/Weld Joint  JointMode=Normal  CompositeWrenchDir=FollowerOnBase  CompositeWrenchFrame=BaseFrame  SenseConstraintForce=off  SenseConstraintTorque=off  SenseTotalForce=on  SenseTotalTorque=off
  HP : PMIOPort  Side=Right
  Upr : PMIOPort  Port=2  Side=Left
  Out Bus Element : Outport  PortName=m  Element=Front
  Out Bus Element1 : Outport  PortName=m  Element=Rear
  wires:
  PS-Simulink Converter/1 -> Out Bus Element/1
  PS-Simulink Converter1/1 -> Out Bus Element1/1
  connections:
  Arm R1/RConn1 -- Arm F1/RConn1 -- Upr/RConn1
  Transform Align UAf UAr1/LConn1 -- Arm F1/LConn1
  Transform Align UAr UAf/RConn1 -- Simscape Bus HP/LConn3 -- Transform Inboard FR Ctr/LConn1
  Transform Align UAf UAr/RConn1 -- Simscape Bus HP/LConn1
  Transform Inboard FR Ctr/RConn1 -- Simscape Bus HP/LConn2
  Simscape Bus HP/RConn1 -- HP/RConn1
  Transform Align UAf UAr/LConn1 -- Arm F2/LConn1
  Transform Align UAf UAr2/RConn1 -- Weld Joint/RConn1
  Arm F2/RConn1 -- Transform Align UAf UAr2/LConn1
  Weld Joint/LConn1 -- Transform Align UAf UAr1/RConn1
  Weld Joint/RConn2 -- PS-Simulink Converter/LConn1
  Arm R1/LConn1 -- Transform Align UAf UAr3/LConn1
  Transform Align UAf UAr4/RConn1 -- Weld Joint1/RConn1
  Weld Joint1/LConn1 -- Transform Align UAf UAr3/RConn1
  Arm R2/RConn1 -- Transform Align UAf UAr4/LConn1
  Arm R2/LConn1 -- Transform Align UAr UAf/LConn1
  Weld Joint1/RConn2 -- PS-Simulink Converter1/LConn1

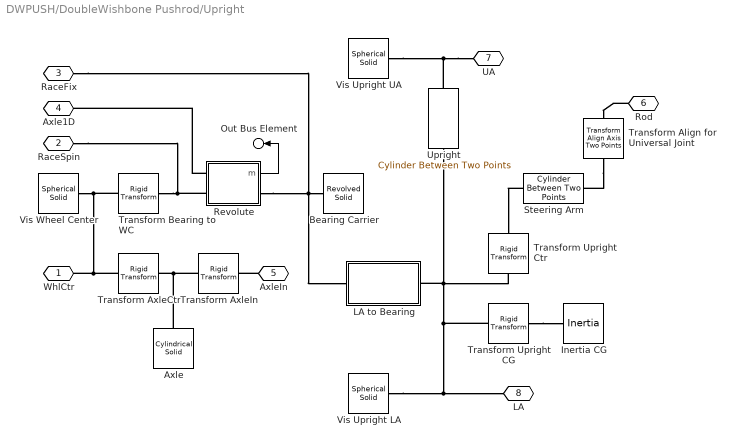
== system DWPUSH/DoubleWishbone Pushrod/Upright ==
  Axle : sm_lib/Body Elements/Cylindrical Solid  CylinderRadius=radius_axle  CylinderRadiusUnits=m  CylinderLength=axle_len  CylinderLengthUnits=m  ExportEntireGeometry=off  InertiaType=CalculateFromGeometry  BasedOnType=Mass  Density=7000  DensityUnits=kg/m^3  Mass=axle_mass  MassUnits=kg  CenterOfMass=[0 0 0]  CenterOfMassUnits=m  MomentsOfInertia=[1 1 1]  MomentsOfInertiaUnits=kg*m^2  ProductsOfInertia=[0 0 0]  ProductsOfInertiaUnits=kg*m^2  GraphicType=FromGeometry  MarkerShape=Sphere  MarkerSize=10  GraphicVisPropType=SimpleVisualProperties  GraphicDiffuseColor=clr_axle  GraphicOpacity=opc_axle  GraphicSpecularColor=[0.5 0.5 0.5 1.0]  GraphicAmbientColor=[0.15 0.15 0.15 1.0]  GraphicEmissiveColor=[0.0 0.0 0.0 1.0]  GraphicShininess=75  DoExposeReferenceFrame=on  SerializedFrames=<Frames/>
  Bearing Carrier : sm_lib/Body Elements/Revolved Solid  RevolutionCrossSection=[1.2 0.5;1.1 0.5;1.1 -0.5;1.2 -0.5].*[radius_axle 0.05]  RevolutionCrossSectionUnits=m  RevolutionExtent=Full  RevolutionAngle=180  RevolutionAngleUnits=deg  ExportConvexHullGeometry=off  InertiaType=CalculateFromGeometry  BasedOnType=Density  Density=1000  DensityUnits=kg/m^3  Mass=1  MassUnits=kg  CenterOfMass=[0 0 0]  CenterOfMassUnits=m  MomentsOfInertia=[1 1 1]  MomentsOfInertiaUnits=kg*m^2  ProductsOfInertia=[0 0 0]  ProductsOfInertiaUnits=kg*m^2  GraphicType=FromGeometry  MarkerShape=Sphere  MarkerSize=10  GraphicVisPropType=SimpleVisualProperties  GraphicDiffuseColor=clr_upr  GraphicOpacity=0.5  GraphicSpecularColor=[0.5 0.5 0.5 1.0]  GraphicAmbientColor=[0.15 0.15 0.15 1.0]  GraphicEmissiveColor=[0.0 0.0 0.0 1.0]  GraphicShininess=75  DoExposeReferenceFrame=on  SerializedFrames=<Frames/>
  Inertia CG : sm_lib/Body Elements/Inertia  InertiaType=PointMass  Mass=upr_mass  MassUnits=kg  CenterOfMass=[0 0 0]  CenterOfMassUnits=m  MomentsOfInertia=[1 1 1]  MomentsOfInertiaUnits=kg*m^2  ProductsOfInertia=[0 0 0]  ProductsOfInertiaUnits=kg*m^2  GraphicType=Marker  MarkerShape=Inertia  MarkerSize=20  GraphicVisPropType=SimpleVisualProperties  GraphicDiffuseColor=[0.5 0.5 0.5]  GraphicOpacity=0  GraphicSpecularColor=[0.5 0.5 0.5 1.0]  GraphicAmbientColor=[0.15 0.15 0.15 1.0]  GraphicEmissiveColor=[0.0 0.0 0.0 1.0]  GraphicShininess=75
  LA to Bearing : Subsystem
  Revolute : Subsystem  mask(Revolute Joint with 1D connections){whl_init_spd_jnt=whl_init_spd_upr}
      mask prompts: whl_init_spd_jnt "Initial Wheel Speed (rad/s)"
      mask help: Multibody Revolute Joint with connection to 1D mechanical network. Specify initial speed of Revolute Joint.
      mask Display: image('sm_car_variant_revolute.png')
  Steering Arm : Suspension_Utilities/Cylinder Between Two Points  hp_b=(hp_la_out+0.5*(hp_ua_out-hp_la_out)).*rhs_hp  hp_f=hp_upr_rod.*rhs_hp  Mass=0  clr_solid=clr_upr  opc_solid=opc_upr  rad_solid=radius_upr
      settings: SourceProductName=SmCar - Suspension Utilites
  Transform Align for Universal Joint : Suspension_Utilities/Transform Align Axis Two Points  hp_b=(hp_la_out+0.5*(hp_ua_out-hp_la_out)).*rhs_hp  hp_t=hp_upr_rod.*rhs_hp  popup_f_axis=+Z
      settings: SourceProductName=SmCar - Suspension Utilites
  Transform AxleCtr : sm_lib/Frames and Transforms/Rigid Transform  RotationMethod=None  FollAlignAxisA=+X  BaseAlignAxisA=+Y  FollAlignAxisB=+Y  BaseAlignAxisB=+Z  RotationStandardAxis=+Z  RotationAngle=0  RotationAngleUnits=deg  RotationArbitraryAxis=[0 0 1]  RotationSequenceAxes=FollowerAxes  RotationSequence=XYX  RotationSequenceAngles=[0 0 0]  RotationSequenceAnglesUnits=deg  RotationMatrix=[1 0 0; 0 1 0; 0 0 1]  Quaternion=[1 0 0 0]  TranslationMethod=StandardAxis  TranslationCartesianOffset=[0 0 0]  TranslationCartesianOffsetUnits=m  TranslationStandardAxis=-Z  TranslationStandardOffset=axle_len*rhs_upr/2  TranslationStandardOffsetUnits=m  TranslationROffset=0  TranslationROffsetUnits=m  TranslationThetaOffset=0  TranslationThetaOffsetUnits=deg  TranslationZOffset=0  TranslationZOffsetUnits=m
  Transform AxleIn : sm_lib/Frames and Transforms/Rigid Transform  RotationMethod=None  FollAlignAxisA=+X  BaseAlignAxisA=+Y  FollAlignAxisB=+Y  BaseAlignAxisB=+Z  RotationStandardAxis=+Z  RotationAngle=0  RotationAngleUnits=deg  RotationArbitraryAxis=[0 0 1]  RotationSequenceAxes=FollowerAxes  RotationSequence=XYX  RotationSequenceAngles=[0 0 0]  RotationSequenceAnglesUnits=deg  RotationMatrix=[1 0 0; 0 1 0; 0 0 1]  Quaternion=[1 0 0 0]  TranslationMethod=StandardAxis  TranslationCartesianOffset=[0 0 0]  TranslationCartesianOffsetUnits=m  TranslationStandardAxis=-Z  TranslationStandardOffset=axle_len*rhs_upr/2  TranslationStandardOffsetUnits=m  TranslationROffset=0  TranslationROffsetUnits=m  TranslationThetaOffset=0  TranslationThetaOffsetUnits=deg  TranslationZOffset=0  TranslationZOffsetUnits=m
  Transform Bearing to WC : sm_lib/Frames and Transforms/Rigid Transform  RotationMethod=None  FollAlignAxisA=+X  BaseAlignAxisA=+Y  FollAlignAxisB=+Y  BaseAlignAxisB=+Z  RotationStandardAxis=+Z  RotationAngle=0  RotationAngleUnits=deg  RotationArbitraryAxis=[0 0 1]  RotationSequenceAxes=FollowerAxes  RotationSequence=XYX  RotationSequenceAngles=[0 0 0]  RotationSequenceAnglesUnits=deg  RotationMatrix=[1 0 0; 0 1 0; 0 0 1]  Quaternion=[1 0 0 0]  TranslationMethod=StandardAxis  TranslationCartesianOffset=[0 0 0]  TranslationCartesianOffsetUnits=m  TranslationStandardAxis=+Z  TranslationStandardOffset=axle_whlc_to_bearing*rhs_upr  TranslationStandardOffsetUnits=m  TranslationROffset=0  TranslationROffsetUnits=m  TranslationThetaOffset=0  TranslationThetaOffsetUnits=deg  TranslationZOffset=0  TranslationZOffsetUnits=m
  Transform Upright CG : sm_lib/Frames and Transforms/Rigid Transform  RotationMethod=None  FollAlignAxisA=+X  BaseAlignAxisA=+Y  FollAlignAxisB=+Y  BaseAlignAxisB=+Z  RotationStandardAxis=+Z  RotationAngle=0.0  RotationAngleUnits=deg  RotationArbitraryAxis=[0 0 1]  RotationSequenceAxes=FollowerAxes  RotationSequence=XYX  RotationSequenceAngles=[0 0 0]  RotationSequenceAnglesUnits=deg  RotationMatrix=[1 0 0; 0 1 0; 0 0 1]  Quaternion=[1 0 0 0]  TranslationMethod=Cartesian  TranslationCartesianOffset=(hp_upr_cg-hp_la_out) .* [1, rhs_upr, 1]  TranslationCartesianOffsetUnits=m  TranslationStandardAxis=+Z  TranslationStandardOffset=0  TranslationStandardOffsetUnits=m  TranslationROffset=0  TranslationROffsetUnits=m  TranslationThetaOffset=0  TranslationThetaOffsetUnits=deg  TranslationZOffset=0  TranslationZOffsetUnits=m
  Transform Upright Ctr : sm_lib/Frames and Transforms/Rigid Transform  RotationMethod=None  FollAlignAxisA=+X  BaseAlignAxisA=+Y  FollAlignAxisB=+Y  BaseAlignAxisB=+Z  RotationStandardAxis=+Z  RotationAngle=0.0  RotationAngleUnits=deg  RotationArbitraryAxis=[0 0 1]  RotationSequenceAxes=FollowerAxes  RotationSequence=XYX  RotationSequenceAngles=[0 0 0]  RotationSequenceAnglesUnits=deg  RotationMatrix=[1 0 0; 0 1 0; 0 0 1]  Quaternion=[1 0 0 0]  TranslationMethod=Cartesian  TranslationCartesianOffset=0.5*(hp_ua_out-hp_la_out).*rhs_hp  TranslationCartesianOffsetUnits=m  TranslationStandardAxis=+Z  TranslationStandardOffset=0  TranslationStandardOffsetUnits=m  TranslationROffset=0  TranslationROffsetUnits=m  TranslationThetaOffset=0  TranslationThetaOffsetUnits=deg  TranslationZOffset=0  TranslationZOffsetUnits=m
  Upright : Suspension_Utilities/Cylinder Between Two Points  hp_b=hp_la_out.*rhs_hp  hp_f=hp_ua_out.*rhs_hp  Mass=0  clr_solid=clr_upr  opc_solid=opc_upr  rad_solid=radius_upr
      settings: SourceProductName=SmCar - Suspension Utilites
  Vis Upright LA : sm_lib/Body Elements/Spherical Solid  SphereRadius=size_conn_upr  SphereRadiusUnits=m  ExportEntireGeometry=off  InertiaType=PointMass  BasedOnType=Density  Density=0  DensityUnits=kg/m^3  Mass=0  MassUnits=kg  CenterOfMass=[0 0 0]  CenterOfMassUnits=m  MomentsOfInertia=[1 1 1]  MomentsOfInertiaUnits=kg*m^2  ProductsOfInertia=[0 0 0]  ProductsOfInertiaUnits=kg*m^2  GraphicType=FromGeometry  MarkerShape=Sphere  MarkerSize=10  GraphicVisPropType=SimpleVisualProperties  GraphicDiffuseColor=clr_conn_upr  GraphicOpacity=opc_conn_upr  GraphicSpecularColor=[0.5 0.5 0.5 1.0]  GraphicAmbientColor=[0.15 0.15 0.15 1.0]  GraphicEmissiveColor=[0.0 0.0 0.0 1.0]  GraphicShininess=75  DoExposeReferenceFrame=on  SerializedFrames=<Frames/>
  Vis Upright UA : sm_lib/Body Elements/Spherical Solid  SphereRadius=size_conn_upr  SphereRadiusUnits=m  ExportEntireGeometry=off  InertiaType=PointMass  BasedOnType=Density  Density=0  DensityUnits=kg/m^3  Mass=0  MassUnits=kg  CenterOfMass=[0 0 0]  CenterOfMassUnits=m  MomentsOfInertia=[1 1 1]  MomentsOfInertiaUnits=kg*m^2  ProductsOfInertia=[0 0 0]  ProductsOfInertiaUnits=kg*m^2  GraphicType=FromGeometry  MarkerShape=Sphere  MarkerSize=10  GraphicVisPropType=SimpleVisualProperties  GraphicDiffuseColor=clr_conn_upr  GraphicOpacity=opc_conn_upr  GraphicSpecularColor=[0.5 0.5 0.5 1.0]  GraphicAmbientColor=[0.15 0.15 0.15 1.0]  GraphicEmissiveColor=[0.0 0.0 0.0 1.0]  GraphicShininess=75  DoExposeReferenceFrame=on  SerializedFrames=<Frames/>
  Vis Wheel Center : sm_lib/Body Elements/Spherical Solid  SphereRadius=size_conn_upr  SphereRadiusUnits=m  ExportEntireGeometry=off  InertiaType=PointMass  BasedOnType=Density  Density=0  DensityUnits=kg/m^3  Mass=0  MassUnits=kg  CenterOfMass=[0 0 0]  CenterOfMassUnits=m  MomentsOfInertia=[1 1 1]  MomentsOfInertiaUnits=kg*m^2  ProductsOfInertia=[0 0 0]  ProductsOfInertiaUnits=kg*m^2  GraphicType=FromGeometry  MarkerShape=Sphere  MarkerSize=10  GraphicVisPropType=SimpleVisualProperties  GraphicDiffuseColor=clr_conn_upr  GraphicOpacity=opc_conn_upr  GraphicSpecularColor=[0.5 0.5 0.5 1.0]  GraphicAmbientColor=[0.15 0.15 0.15 1.0]  GraphicEmissiveColor=[0.0 0.0 0.0 1.0]  GraphicShininess=75  DoExposeReferenceFrame=on  SerializedFrames=<Frames/>
  WhlCtr : PMIOPort  Side=Left
  RaceSpin : PMIOPort  Port=2  Side=Left
  RaceFix : PMIOPort  Port=3  Side=Left
  Axle1D : PMIOPort  Port=4  Side=Left
  AxleIn : PMIOPort  Port=5  Side=Left
  Rod : PMIOPort  Port=6  Side=Right
  UA : PMIOPort  Port=7  Side=Right
  LA : PMIOPort  Port=8  Side=Right
  Out Bus Element : Outport  VectorParamsAs1DForOutWhenUnconnected=off  PortName=m  Element=Upright
  wires:
  Revolute/1(m) -> Out Bus Element/1
  connections:
  AxleIn/RConn1 -- Transform AxleIn/RConn1
  Transform AxleCtr/RConn1 -- Transform AxleIn/LConn1 -- Axle/RConn1
  Transform Bearing to WC/LConn1 -- Revolute/LConn2 -- RaceSpin/RConn1
  Bearing Carrier/RConn1 -- LA to Bearing/LConn1 -- Revolute/RConn1 -- RaceFix/RConn1
  Transform Align for Universal Joint/LConn1 -- Steering Arm/RConn1
  Rod/RConn1 -- Transform Align for Universal Joint/RConn1
  Steering Arm/LConn1 -- Transform Upright Ctr/RConn1
  Transform Upright CG/RConn1 -- Inertia CG/RConn1
  UA/RConn1 -- Upright/RConn1 -- Vis Upright UA/RConn1
  Vis Upright LA/RConn1 -- Transform Upright CG/LConn1 -- LA to Bearing/RConn1 -- Upright/LConn1 -- Transform Upright Ctr/LConn1 -- LA/RConn1
  Transform Bearing to WC/RConn1 -- Transform AxleCtr/LConn1 -- WhlCtr/RConn1 -- Vis Wheel Center/RConn1
  Revolute/LConn1 -- Axle1D/RConn1
